simulink model "hdlcoder_delays_eml"  (R2026a)
settings: Solver=VariableStepDiscrete  EnableMultiTasking=on
InitFcn:
  | N = 4;
libraries: simulink x6
settings Model: Creator=The MathWorks, Inc.  LastModifiedBy=The MathWorks, Inc.
settings OptimizationCC: InitFltsAndDblsToZero=on
settings DebuggingCC: SaveWithParameterizedLinksMsg=none  UnderspecifiedInitializationDetection=Classic  MultiTaskDSMMsg=warning  MultiTaskCondExecSysMsg=none
settings HardwareCC: ProdHWDeviceType=32-bit Generic  TargetHWDeviceType=32-bit Generic
settings GRTTargetCC: TargetFcnLib=ansi_tfl_tmw.mat  CombineOutputUpdateFcns=off  GRTInterface=on

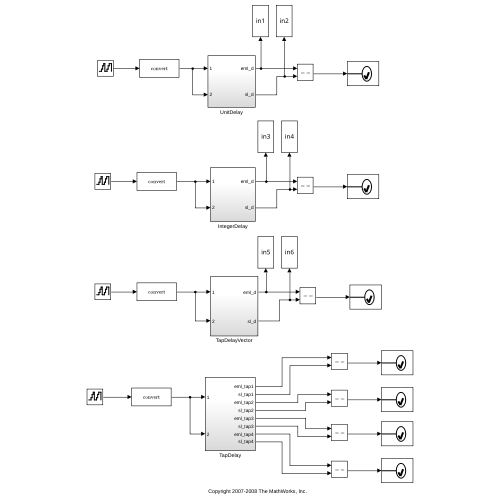
[thumbnail: Simulink's stored preview of the top-level diagram]
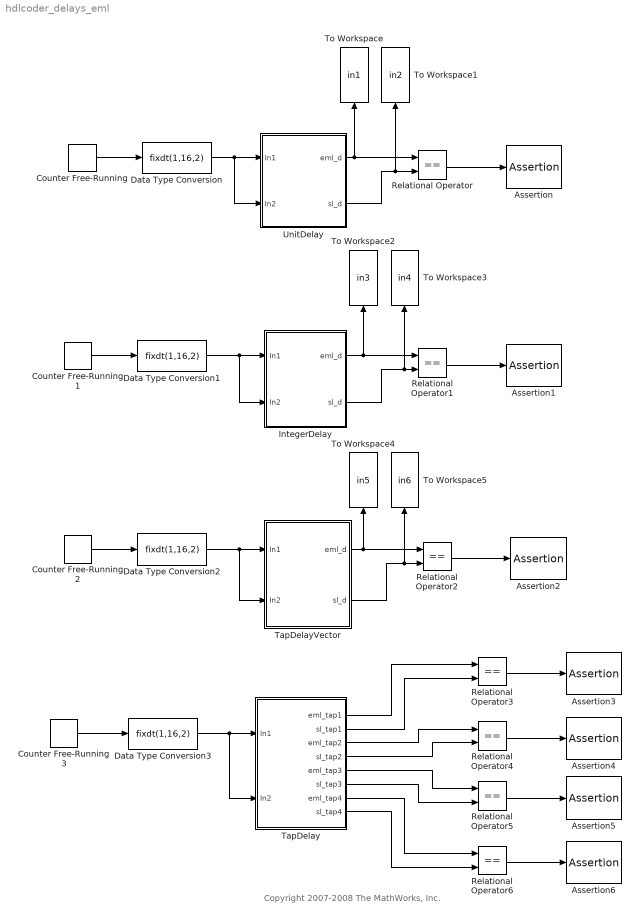
== system hdlcoder_delays_eml ==
  note: Copyright 2007-2008 The MathWorks, Inc.
  Assertion{,1..6} (7 alike) : Assertion
  Counter Free-Running{,1..3} (4 alike) : simulink/Sources/Counter Free-Running  NumBits=16  tsamp=-1
  Data Type Conversion{,1..3} (4 alike) : DataTypeConversion  OutDataTypeStr=fixdt(1,16,2)  SaturateOnIntegerOverflow=off  RndMeth=Floor
  IntegerDelay : Subsystem
  Relational Operator{,1..6} (7 alike) : RelationalOperator  Operator===  OutDataTypeStr=boolean  InputSameDT=off
  TapDelay : Subsystem
  TapDelayVector : Subsystem
  To Workspace : ToWorkspace  VariableName=in1  SampleTime=-1
  To Workspace1 : ToWorkspace  VariableName=in2  SampleTime=-1
  To Workspace2 : ToWorkspace  VariableName=in3  SampleTime=-1
  To Workspace3 : ToWorkspace  VariableName=in4  SampleTime=-1
  To Workspace4 : ToWorkspace  VariableName=in5  SampleTime=-1
  To Workspace5 : ToWorkspace  VariableName=in6  SampleTime=-1
  UnitDelay : Subsystem
  wires:
  Counter Free-Running/1 -> Data Type Conversion/1
  Data Type Conversion/1 -> UnitDelay/1(In1), UnitDelay/2(In2)
  Counter Free-Running1/1 -> Data Type Conversion1/1
  Data Type Conversion1/1 -> IntegerDelay/1(In1), IntegerDelay/2(In2)
  Counter Free-Running2/1 -> Data Type Conversion2/1
  Data Type Conversion2/1 -> TapDelayVector/1(In1), TapDelayVector/2(In2)
  Data Type Conversion3/1 -> TapDelay/1(In1), TapDelay/2(In2)
  UnitDelay/1(eml_d) -> Relational Operator/1, To Workspace/1
  UnitDelay/2(sl_d) -> Relational Operator/2, To Workspace1/1
  Relational Operator/1 -> Assertion/1
  IntegerDelay/1(eml_d) -> Relational Operator1/1, To Workspace2/1
  IntegerDelay/2(sl_d) -> Relational Operator1/2, To Workspace3/1
  Relational Operator1/1 -> Assertion1/1
  TapDelayVector/1(eml_d) -> To Workspace4/1, Relational Operator2/1
  TapDelayVector/2(sl_d) -> Relational Operator2/2, To Workspace5/1
  Relational Operator2/1 -> Assertion2/1
  Relational Operator3/1 -> Assertion3/1
  Relational Operator4/1 -> Assertion4/1
  Relational Operator5/1 -> Assertion5/1
  Relational Operator6/1 -> Assertion6/1
  TapDelay/1(eml_tap1) -> Relational Operator3/1
  TapDelay/2(sl_tap1) -> Relational Operator3/2
  TapDelay/3(eml_tap2) -> Relational Operator4/1
  TapDelay/4(sl_tap2) -> Relational Operator4/2
  TapDelay/5(eml_tap3) -> Relational Operator5/1
  TapDelay/6(sl_tap3) -> Relational Operator5/2
  TapDelay/7(eml_tap4) -> Relational Operator6/1
  TapDelay/8(sl_tap4) -> Relational Operator6/2
  Counter Free-Running3/1 -> Data Type Conversion3/1

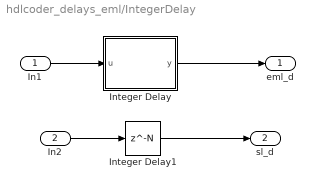
== system hdlcoder_delays_eml/IntegerDelay ==
  In1 : Inport
  In2 : Inport  Port=2
  Integer Delay : MATLAB Function  TreatAsAtomicUnit=on
  Integer Delay1 : Delay  DelayLength=N
  eml_d : Outport
  sl_d : Outport  Port=2
  wires:
  In1/1 -> Integer Delay/1(u)
  Integer Delay/1(y) -> eml_d/1
  In2/1 -> Integer Delay1/1
  Integer Delay1/1 -> sl_d/1

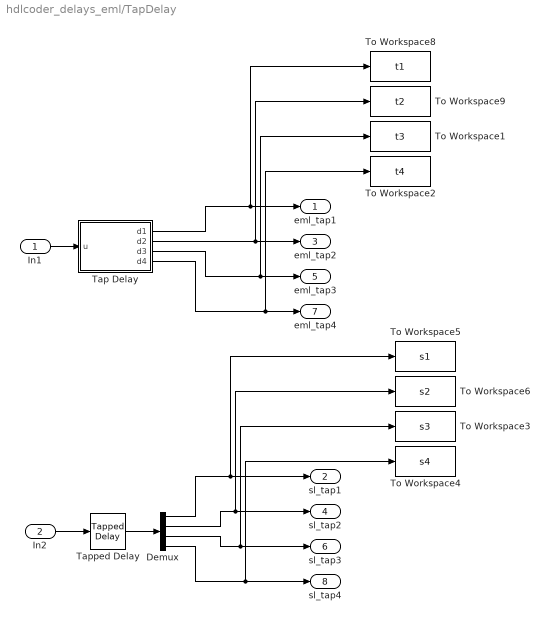
== system hdlcoder_delays_eml/TapDelay ==
  In1 : Inport
  In2 : Inport  Port=2
  Demux : Demux
  Tap Delay : MATLAB Function  TreatAsAtomicUnit=on
  Tapped Delay : simulink/Discrete/Tapped Delay  vinit=0.0  samptime=-1  NumDelays=N  DelayOrder=Oldest  includeCurrent=off
  To Workspace1 : ToWorkspace  VariableName=t3  SampleTime=-1
  To Workspace2 : ToWorkspace  VariableName=t4  SampleTime=-1
  To Workspace3 : ToWorkspace  VariableName=s3  SampleTime=-1
  To Workspace4 : ToWorkspace  VariableName=s4  SampleTime=-1
  To Workspace5 : ToWorkspace  VariableName=s1  SampleTime=-1
  To Workspace6 : ToWorkspace  VariableName=s2  SampleTime=-1
  To Workspace8 : ToWorkspace  VariableName=t1  SampleTime=-1
  To Workspace9 : ToWorkspace  VariableName=t2  SampleTime=-1
  eml_tap1 : Outport
  sl_tap1 : Outport  Port=2
  eml_tap2 : Outport  Port=3
  sl_tap2 : Outport  Port=4
  eml_tap3 : Outport  Port=5
  sl_tap3 : Outport  Port=6
  eml_tap4 : Outport  Port=7
  sl_tap4 : Outport  Port=8
  wires:
  In1/1 -> Tap Delay/1(u)
  In2/1 -> Tapped Delay/1
  Tapped Delay/1 -> Demux/1
  Demux/1 -> sl_tap1/1, To Workspace5/1
  Demux/2 -> sl_tap2/1, To Workspace6/1
  Demux/3 -> sl_tap3/1, To Workspace3/1
  Demux/4 -> sl_tap4/1, To Workspace4/1
  Tap Delay/1(d1) -> eml_tap1/1, To Workspace8/1
  Tap Delay/2(d2) -> eml_tap2/1, To Workspace9/1
  Tap Delay/3(d3) -> eml_tap3/1, To Workspace1/1
  Tap Delay/4(d4) -> eml_tap4/1, To Workspace2/1

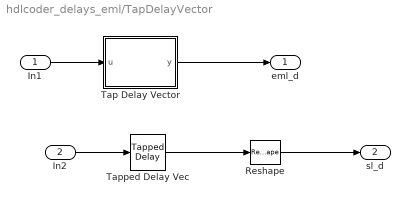
== system hdlcoder_delays_eml/TapDelayVector ==
  In1 : Inport
  In2 : Inport  Port=2
  Reshape : Reshape  OutputDimensionality=Row vector (2-D)
  Tap Delay Vector : MATLAB Function  TreatAsAtomicUnit=on
  Tapped Delay Vec : simulink/Discrete/Tapped Delay  vinit=0.0  samptime=-1  NumDelays=N  DelayOrder=Oldest  includeCurrent=off
  eml_d : Outport
  sl_d : Outport  Port=2
  wires:
  In1/1 -> Tap Delay Vector/1(u)
  Tap Delay Vector/1(y) -> eml_d/1
  In2/1 -> Tapped Delay Vec/1
  Tapped Delay Vec/1 -> Reshape/1
  Reshape/1 -> sl_d/1

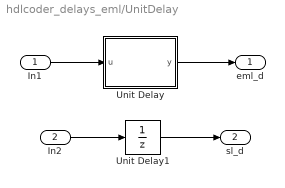
== system hdlcoder_delays_eml/UnitDelay ==
  In1 : Inport
  In2 : Inport  Port=2
  Unit Delay : MATLAB Function  TreatAsAtomicUnit=on
  Unit Delay1 : UnitDelay
  eml_d : Outport
  sl_d : Outport  Port=2
  wires:
  In1/1 -> Unit Delay/1(u)
  Unit Delay/1(y) -> eml_d/1
  In2/1 -> Unit Delay1/1
  Unit Delay1/1 -> sl_d/1

== matlab function hdlcoder_delays_eml/IntegerDelay/Integer Delay ==
  settings: fimath=|
      | fimath(...
      | 'RoundMode', 'floor',...
      | 'OverflowMode', 'wrap',...
      | 'ProductMode', 'FullPrecision', 'ProductWordLength', 32,...
      | 'SumMode', 'FullPrecision', 'SumWordLength', 32,...
      | 'CastBeforeSum', true)
  data: u input; y output; N parameter
function y = fcn(u, N)

% The Integer Delay block delays its input by N sample periods. 
% The block accepts one input and generates one output, both of which
% can be scalar or vector. If the input is a vector, all elements of the 
% vector are delayed by the same sample period.

% In this example N is hardwired as 4; This function behaves as Integer 
% delay block and delays inputs by 4 sample hits.

persistent u_d;
if isempty(u_d)
	% defines initial value driven by integer delay 
    % from time step 0 to time step N-1
    u_d = fi(zeros(1,N), numerictype(u), fimath(u));
end

y = u_d(N);

u_d = [u, u_d(1:N-1)];

== matlab function hdlcoder_delays_eml/TapDelay/Tap Delay ==
  settings: fimath=|
      | fimath(...
      | 'RoundMode', 'floor',...
      | 'OverflowMode', 'wrap',...
      | 'ProductMode', 'FullPrecision', 'ProductWordLength', 32,...
      | 'SumMode', 'FullPrecision', 'SumWordLength', 32,...
      | 'CastBeforeSum', true)
  data: u input; d1 output; d2 output; d3 output; d4 output
function [d1, d2, d3, d4] = fcn(u)
%The Tapped Delay function delays its input by the specified number 
% of sample periods, and outputs all the delayed versions.

% In this example the number of output taps is hardwired to 4.

persistent u_d;
if isempty(u_d)
    % defines initial value driven by integer delay 
    % from time step 0 to time step N-1
    u_d = fi(zeros(1,4), numerictype(u), fimath(u));
end

d1 = u_d(1);
d2 = u_d(2);
d3 = u_d(3);
d4 = u_d(4);

u_d = [u_d(2:4), u];

== matlab function hdlcoder_delays_eml/TapDelayVector/Tap Delay Vector ==
  settings: fimath=|
      | fimath(...
      | 'RoundMode', 'floor',...
      | 'OverflowMode', 'wrap',...
      | 'ProductMode', 'FullPrecision', 'ProductWordLength', 32,...
      | 'SumMode', 'FullPrecision', 'SumWordLength', 32,...
      | 'CastBeforeSum', true)
  data: u input; y output
function y = fcn(u)
% The Tapped Delay function delays its input by the specified number 
% of sample periods, and outputs all the delayed versions in a vector
% form.

% In this example N is hardwired to 4.

persistent u_d;
if isempty(u_d)
    u_d = fi(zeros(1,4), numerictype(u), fimath(u));
end

y = u_d;

u_d = [u_d(2), u_d(3), u_d(4), u];

== matlab function hdlcoder_delays_eml/UnitDelay/Unit Delay ==
  settings: fimath=|
      | fimath(...
      | 'RoundMode', 'floor',...
      | 'OverflowMode', 'wrap',...
      | 'ProductMode', 'FullPrecision', 'ProductWordLength', 32,...
      | 'SumMode', 'FullPrecision', 'SumWordLength', 32,...
      | 'CastBeforeSum', true)
  data: u input; y output
function y = fcn(u)
% Complex unit delay

% The Unit Delay block delays its input by the specified sample period.
% The block accepts one input and generates one output, which can
% be either both scalar or both vector. If the input is a vector, 
% all elements of the vector are delayed by the same sample period.
%
% You specify the block output for the first sampling period with the 
% Initial value to the persistent variable.
%

% y is same as u delayed by one sample period.

% output of this block at the first sample hit is decided by the initial 
% value of this persistent variable.

persistent u_d;
if isempty(u_d)
    % defines initial value driven by unit delay at time step 0
    u_d = fi(0, numerictype(u), fimath(u));
end

% return delayed input from last sample time hit
y = u_d;

% store the current input to be used later
u_d = u;
